simulink model "Simple_Pendulumn_v2"  (R2021b)
settings: Solver=VariableStepAuto  StartTime=0.0  StopTime=30  MaxStep=0.001  RelTol=1e-3
model workspace (MAT data in the model file):
  b = 0.05
  g = 9.81
  l = 0.5
  m = 0.2
undefined symbols (not defined in the file): X, Y, Z
libraries: sm_lib x8, nesl_utility x3
settings Model: Creator=Sandun Sudasingha  LastModifiedBy=Sandun Sudasinghe
settings SolverCC: AlgebraicLoopSolver=TrustRegion
settings DataIOCC: ReturnWorkspaceOutputs=off
settings DebuggingCC: SFMachineParentedDataDiag=warning  ArithmeticOperatorsInVariantConditions=warning
settings SFSimCC: SimUseLocalCustomCode=off  CustomCodeUndefinedFunction=UseInterfaceOnly
settings RTWCC: RTWUseLocalCustomCode=off

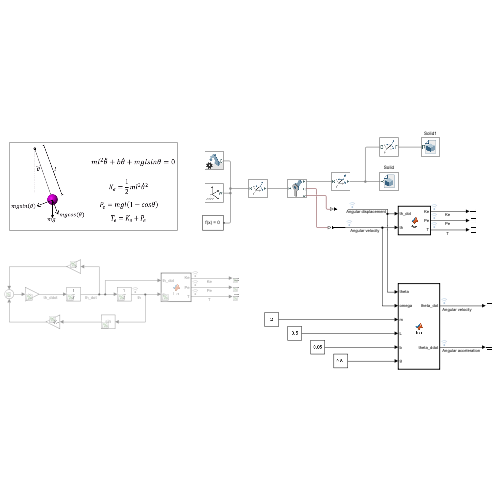
[thumbnail: Simulink's stored preview of the top-level diagram]
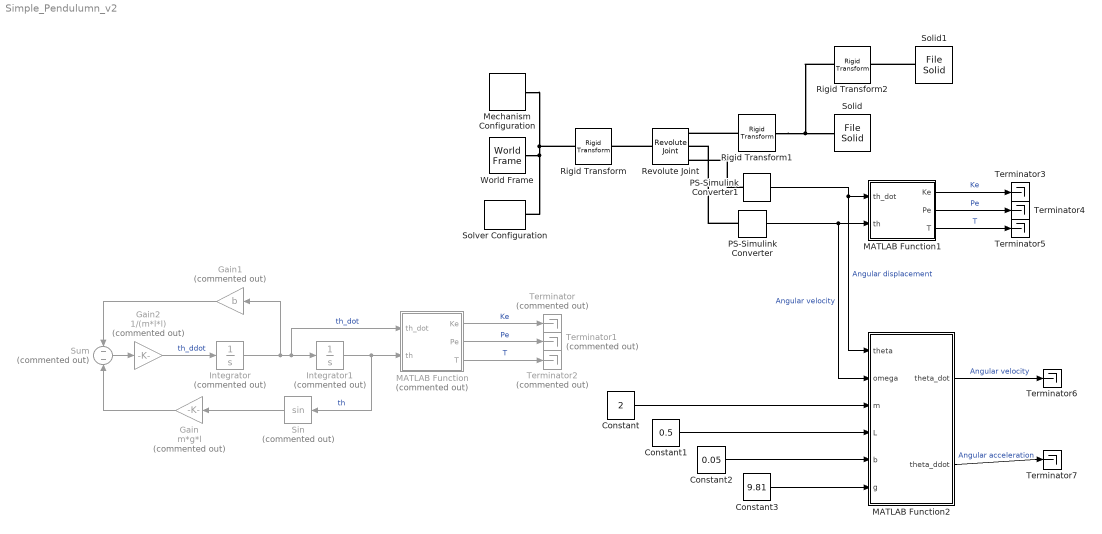
== system Simple_Pendulumn_v2 ==
  Constant : Constant  Value=2
  Constant1 : Constant  Value=0.5
  Constant2 : Constant  Value=0.05
  Constant3 : Constant  Value=9.81
  Gain : Gain  Commented=on  Gain=m*g*l
  Gain1 : Gain  Commented=on  Gain=b
  Gain2 : Gain  Commented=on  Gain=1/(m*l*l)
  Integrator : Integrator  Commented=on
  Integrator1 : Integrator  Commented=on  InitialCondition=0.5
  MATLAB Function : MATLAB Function  Commented=on  TreatAsAtomicUnit=on
  MATLAB Function1 : MATLAB Function  TreatAsAtomicUnit=on
  MATLAB Function2 : MATLAB Function  TreatAsAtomicUnit=on
  Mechanism Configuration : sm_lib/Utilities/Mechanism Configuration  UniformGravity=Constant  GravityVector=[0 0 -9.81]  GravityUnits=m/s^2  LinearizationDelta=0.001  JointModeTransitionNonlinearIterations=2
  PS-Simulink Converter : nesl_utility/PS-Simulink Converter  PhysicalDomain=network_engine_domain  SubClassName=ps_output  LeftPortType=input  RightPortType=output  PseudoPeriodic=off  Frequencies=[]  Unit=1  AffineConversion=off
      settings: SourceProductBaseCode=PW,SS
  PS-Simulink Converter1 : nesl_utility/PS-Simulink Converter  PhysicalDomain=network_engine_domain  SubClassName=ps_output  LeftPortType=input  RightPortType=output  PseudoPeriodic=off  Frequencies=[]  Unit=1  AffineConversion=off
      settings: SourceProductBaseCode=PW,SS
  Revolute Joint : sm_lib/Joints/Revolute Joint  JointMode=Normal  SenseConstraintForce=off  SenseConstraintForceX=off  SenseConstraintForceY=off  SenseConstraintForceZ=off  SenseConstraintTorque=off  SenseConstraintTorqueX=off  SenseConstraintTorqueY=off  SenseConstraintTorqueZ=off  SenseTotalForce=off  SenseTotalForceX=off  SenseTotalForceY=off  SenseTotalForceZ=off  SenseTotalTorque=off  SenseTotalTorqueX=off  SenseTotalTorqueY=off  SenseTotalTorqueZ=off  CompositeWrenchDir=FollowerOnBase  CompositeWrenchFrame=BaseFrame  EquilibriumPosition=0  EquilibriumPositionUnits=deg  SpringStiffness=0  SpringStiffnessUnits=N*m/deg  DampingCoefficient=b  DampingCoefficientUnits=N*m/(rad/s)  TorqueActuationMode=NoTorque  MotionActuationMode=ComputedMotion  SensePosition=on  SenseVelocity=on  SenseAcceleration=off  SenseTorqueForce=off  SenseLowerLimitTorqueForce=off  SenseUpperLimitTorqueForce=off  LowerLimitSpecify=off  LowerLimitBound=-90  LowerLimitBoundUnits=deg  LowerLimitStiffness=1e4  LowerLimitStiffnessUnits=N*m/deg  LowerLimitDamping=10  LowerLimitDampingUnits=N*m/(deg/s)  LowerLimitTransitionRegionWidth=0.1  LowerLimitTransitionRegionWidthUnits=deg  UpperLimitSpecify=off  UpperLimitBound=90  UpperLimitBoundUnits=deg  UpperLimitStiffness=1e4  UpperLimitStiffnessUnits=N*m/deg  UpperLimitDamping=10  UpperLimitDampingUnits=N*m/(deg/s)  UpperLimitTransitionRegionWidth=0.1  UpperLimitTransitionRegionWidthUnits=deg  PositionTargetSpecify=on  PositionTargetPriority=High  PositionTargetValue=0.5  PositionTargetValueUnits=rad  VelocityTargetSpecify=off  VelocityTargetPriority=High  VelocityTargetValue=0  VelocityTargetValueUnits=deg/s
  Rigid Transform : sm_lib/Frames and Transforms/Rigid Transform  TranslationMethod=None  TranslationStandardOffset=0  TranslationLengthUnit=m  TranslationStandardAxis=+Z  TranslationCartesianOffset=[0 0 0]  TranslationROffset=0  TranslationROffsetUnits=m  TranslationZOffset=0  TranslationZOffsetUnits=m  TranslationThetaOffset=0  TranslationThetaOffsetUnits=deg  RotationMethod=StandardAxis  RotationAngleUnits=deg  RotationStandardAxis=+X  RotationAngle=90  RotationArbitraryAxis=[0 0 1]  FollAlignAxisA=+X  BaseAlignAxisA=+Y  FollAlignAxisB=+Y  BaseAlignAxisB=+Z  RotationSequenceAxes=FollowerAxes  RotationSequence=XYX  RotationSequenceAngles=[0 0 0]  RotationSequenceAnglesUnits=deg  RotationMatrix=[1 0 0; 0 1 0; 0 0 1]
  Rigid Transform1 : sm_lib/Frames and Transforms/Rigid Transform  TranslationMethod=StandardAxis  TranslationStandardOffset=l/2  TranslationLengthUnit=m  TranslationStandardAxis=-Y  TranslationCartesianOffset=[0 0 0]  TranslationROffset=0  TranslationROffsetUnits=m  TranslationZOffset=0  TranslationZOffsetUnits=m  TranslationThetaOffset=0  TranslationThetaOffsetUnits=deg  RotationMethod=None  RotationAngleUnits=deg  RotationStandardAxis=+Z  RotationAngle=0.0  RotationArbitraryAxis=[0 0 1]  FollAlignAxisA=+X  BaseAlignAxisA=+Y  FollAlignAxisB=+Y  BaseAlignAxisB=+Z  RotationSequenceAxes=FollowerAxes  RotationSequence=XYX  RotationSequenceAngles=[0 0 0]  RotationSequenceAnglesUnits=deg  RotationMatrix=[1 0 0; 0 1 0; 0 0 1]
  Rigid Transform2 : sm_lib/Frames and Transforms/Rigid Transform  TranslationMethod=StandardAxis  TranslationStandardOffset=l/2  TranslationLengthUnit=m  TranslationStandardAxis=-Y  TranslationCartesianOffset=[0 0 0]  TranslationROffset=0  TranslationROffsetUnits=m  TranslationZOffset=0  TranslationZOffsetUnits=m  TranslationThetaOffset=0  TranslationThetaOffsetUnits=deg  RotationMethod=None  RotationAngleUnits=deg  RotationStandardAxis=+Z  RotationAngle=0.0  RotationArbitraryAxis=[0 0 1]  FollAlignAxisA=+X  BaseAlignAxisA=+Y  FollAlignAxisB=+Y  BaseAlignAxisB=+Z  RotationSequenceAxes=FollowerAxes  RotationSequence=XYX  RotationSequenceAngles=[0 0 0]  RotationSequenceAnglesUnits=deg  RotationMatrix=[1 0 0; 0 1 0; 0 0 1]
  Sin : Trigonometry  Commented=on
  Solid : sm_lib/Body Elements/File Solid  ExtGeomFileName=C:\3 - OTHERS\Mine\Simple Pendumn Project\Solidworks\Part1.STEP  UnitType=FromFile  ExtGeomFileUnits=m  StepReaderType=OCC  ExportConvexHullGeometry=off  InertiaType=CalculateFromGeometry  Mass=0  MassUnits=kg  CenterOfMass=[0 0 0]  CenterOfMassUnits=m  MomentsOfInertia=[1 1 1]  MomentsOfInertiaUnits=kg*m^2  ProductsOfInertia=[0 0 0]  ProductsOfInertiaUnits=kg*m^2  BasedOnType=Mass  Density=1000  DensityUnits=kg/m^3  DoExposeReferenceFrame=on  SerializedFrames=<Frames/>  GraphicType=FromGeometry  MarkerShape=Sphere  MarkerSize=10  GraphicVisPropType=SimpleVisualProperties  GraphicDiffuseColor=[0.5 0.5 0.5]  GraphicSpecularColor=[0.5 0.5 0.5 1.0]  GraphicAmbientColor=[0.15 0.15 0.15 1.0]  GraphicEmissiveColor=[0.0 0.0 0.0 1.0]  GraphicShininess=75  GraphicOpacity=1.0
  Solid1 : sm_lib/Body Elements/File Solid  ExtGeomFileName=C:\3 - OTHERS\Mine\Simple Pendumn Project\Solidworks\Part2.STEP  UnitType=FromFile  ExtGeomFileUnits=m  StepReaderType=OCC  ExportConvexHullGeometry=off  InertiaType=CalculateFromGeometry  Mass=2  MassUnits=kg  CenterOfMass=[0 0 0]  CenterOfMassUnits=m  MomentsOfInertia=[1 1 1]  MomentsOfInertiaUnits=kg*m^2  ProductsOfInertia=[0 0 0]  ProductsOfInertiaUnits=kg*m^2  BasedOnType=Mass  Density=1000  DensityUnits=kg/m^3  DoExposeReferenceFrame=on  SerializedFrames=<Frames/>  GraphicType=FromGeometry  MarkerShape=Sphere  MarkerSize=10  GraphicVisPropType=SimpleVisualProperties  GraphicDiffuseColor=[0.1 0.3 0.6]  GraphicSpecularColor=[0.5 0.5 0.5 1.0]  GraphicAmbientColor=[0.15 0.15 0.15 1.0]  GraphicEmissiveColor=[0.0 0.0 0.0 1.0]  GraphicShininess=75  GraphicOpacity=1.0
  Solver Configuration : nesl_utility/Solver Configuration  PhysicalDomain=network_engine_domain  SubClassName=solver  LeftPortType=input  RightPortType=generic  Tones=[]  Harmonics=[]  SimulateNoise=off  Profile=off  UseLocalSampling=off  EnableSwitchedLinearOptims=on  FrequencyDomain=off  UseCCode=off  RelTol=0.001  AbsTol=1e-06  MinStep=1e-09  ToWorkspace=off  RevertToSquareIcSolve=off  NumHomotopyIterations=100  PhasorMode=off  PhasorModeNumHarmonics=1  DoDC=off  ResidualTolerance=1e-09  UseLocalSolver=off  LocalSolverChoice=NE_BACKWARD_EULER_ADVANCER  LocalSolverSampleTime=0.001  DoFixedCost=off  MaxNonlinIter=3  MaxModeIter=2  ComputeImpulses=off  ImpulseIterations=2  LinearAlgebra=Sparse  EquationFormulation=NE_TIME_EF  DelaysMemoryBudget=1024  AutomaticFiltering=on  FilteringTimeConstant=0.001  PartitionStorageMethod=AS_NEEDED  PartitionMemoryBudget=1024  PartitionMethod=FAST
      settings: SourceProductBaseCode=PW,SS
  Sum : Sum  Commented=on  Inputs=-|-
  Terminator : Terminator  Commented=on
  Terminator1 : Terminator  Commented=on
  Terminator2 : Terminator  Commented=on
  Terminator{3..7} (5 alike) : Terminator
  World Frame : sm_lib/Frames and Transforms/World Frame
  wires:
  Integrator/1 -> Gain1/1, MATLAB Function/1(th_dot), Integrator1/1  "th_dot"
  Integrator1/1 -> MATLAB Function/2(th), Sin/1  "th"
  Sin/1 -> Gain/1
  Gain1/1 -> Sum/1
  Gain/1 -> Sum/2
  Gain2/1 -> Integrator/1  "th_ddot"
  Sum/1 -> Gain2/1
  MATLAB Function/1(Ke) -> Terminator/1  "Ke"
  MATLAB Function/3(T) -> Terminator2/1  "T"
  MATLAB Function/2(Pe) -> Terminator1/1  "Pe"
  MATLAB Function1/1(Ke) -> Terminator3/1  "Ke"
  MATLAB Function1/3(T) -> Terminator5/1  "T"
  MATLAB Function1/2(Pe) -> Terminator4/1  "Pe"
  PS-Simulink Converter1/1 -> MATLAB Function2/1(theta), MATLAB Function1/1(th_dot)  "Angular displacement"
  PS-Simulink Converter/1 -> MATLAB Function2/2(omega), MATLAB Function1/2(th)  "Angular velocity"
  Constant/1 -> MATLAB Function2/3(m)
  Constant1/1 -> MATLAB Function2/4(L)
  Constant2/1 -> MATLAB Function2/5(b)
  Constant3/1 -> MATLAB Function2/6(g)
  MATLAB Function2/1(theta_dot) -> Terminator6/1  "Angular velocity"
  MATLAB Function2/2(theta_ddot) -> Terminator7/1  "Angular acceleration"
  connections:
  Mechanism Configuration/RConn1 -- Rigid Transform/LConn1 -- World Frame/RConn1 -- Solver Configuration/RConn1
  Revolute Joint/LConn1 -- Rigid Transform/RConn1
  Rigid Transform1/LConn1 -- Revolute Joint/RConn1
  Rigid Transform1/RConn1 -- Solid/RConn1 -- Rigid Transform2/LConn1
  Solid1/RConn1 -- Rigid Transform2/RConn1
  PS-Simulink Converter/LConn1 -- Revolute Joint/RConn2
  PS-Simulink Converter1/LConn1 -- Revolute Joint/RConn3

== matlab function Simple_Pendulumn_v2/MATLAB Function1 ==
  data: Ke output; Pe output; T output; th_dot input; th input; m parameter; g parameter; l parameter
function [Ke, Pe, T] = fcn(th_dot, th, m, g, l)

Ke = 0.5*m*l^2*th_dot^2;
Pe = m*g*l*(1-cos(th));
T = Ke + Pe;

== matlab function Simple_Pendulumn_v2/MATLAB Function ==
  data: Ke output; Pe output; T output; th_dot input; th input; m parameter; g parameter; l parameter
function [Ke, Pe, T] = fcn(th_dot, th, m, g, l)

Ke = 0.5*m*l^2*th_dot^2;
Pe = m*g*l*(1-cos(th));
T = Ke + Pe;

== matlab function Simple_Pendulumn_v2/MATLAB Function2 ==
  data: theta_dot output; theta_ddot output; theta input; omega input; m input; L input; b input; g input

function [theta_dot, theta_ddot] = fcn(theta, omega, m, L, b, g)
% Simple Pendulum - Nonlinear Mathematical Model
% With viscous damping

% Angular velocity
theta_dot = omega;

% Angular acceleration
theta_ddot = -(b/(m*L^2))*omega - (g/L)*sin(theta);

end
